simulink model "SigmoidSlidingModeObserver"  (R2026b)
settings: Solver=VariableStepAuto
PostLoadFcn:
  | addpath(fullfile(fileparts(get_param(bdroot,'FileName')),'..','build_process'));initialize_sigmoid_smo_paths();
undefined symbols (not defined in the file or in its folder): sigmoid_smo_parameters, sigmoid_smo_pll_parameters
libraries: AngleTracking x1
settings Model: Creator=24322  LastModifiedBy=24322

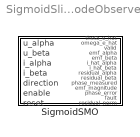
== system SigmoidSlidingModeObserver ==
  SigmoidSMO : Subsystem  mask{cfg=sigmoid_smo_parameters(), trackerCfg=sigmoid_smo_pll_parameters()}
      mask prompts: cfg "Sigmoid SMO configuration"; trackerCfg "PLL configuration"

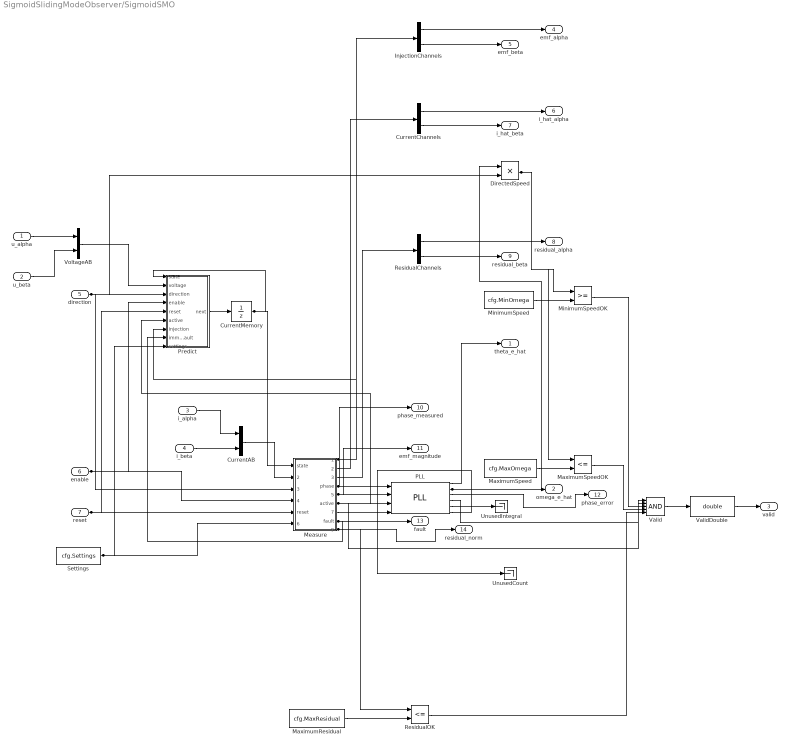
== system SigmoidSlidingModeObserver/SigmoidSMO ==
  u_alpha : Inport  SampleTime=cfg.Ts
  u_beta : Inport  Port=2  SampleTime=cfg.Ts
  i_alpha : Inport  Port=3  SampleTime=cfg.Ts
  i_beta : Inport  Port=4  SampleTime=cfg.Ts
  direction : Inport  Port=5  SampleTime=cfg.Ts
  enable : Inport  Port=6  SampleTime=cfg.Ts
  reset : Inport  Port=7  SampleTime=cfg.Ts
  CurrentAB : Mux  Inputs=2
  CurrentChannels : Demux  Outputs=2
  CurrentMemory : UnitDelay  InitialCondition=zeros(4,1)  SampleTime=cfg.Ts
  DirectedSpeed : Product  Inputs=**
  InjectionChannels : Demux  Outputs=2
  MaximumResidual : Constant  Value=cfg.MaxResidual
  MaximumSpeed : Constant  Value=cfg.MaxOmega
  MaximumSpeedOK : RelationalOperator  Operator=<=  OutDataTypeStr=boolean  RndMeth=Simplest  InputSameDT=off
  Measure : MATLAB Function  TreatAsAtomicUnit=on
  MinimumSpeed : Constant  Value=cfg.MinOmega
  MinimumSpeedOK : RelationalOperator  OutDataTypeStr=boolean  RndMeth=Simplest  InputSameDT=off
  PLL : AngleTracking/PLL  pllCfg=trackerCfg
  Predict : MATLAB Function  TreatAsAtomicUnit=on
  ResidualChannels : Demux  Outputs=2
  ResidualOK : RelationalOperator  Operator=<=  OutDataTypeStr=boolean  RndMeth=Simplest  InputSameDT=off
  Settings : Constant  Value=cfg.Settings
  UnusedCount : Terminator
  UnusedIntegral : Terminator
  Valid : Logic  Inputs=5  IconShape=distinctive  AllPortsSameDT=off  OutDataTypeStr=boolean
  ValidDouble : DataTypeConversion  OutDataTypeStr=double  SaturateOnIntegerOverflow=off  RndMeth=Floor
  VoltageAB : Mux  Inputs=2
  theta_e_hat : Outport
  omega_e_hat : Outport  Port=2
  valid : Outport  Port=3
  emf_alpha : Outport  Port=4
  emf_beta : Outport  Port=5
  i_hat_alpha : Outport  Port=6
  i_hat_beta : Outport  Port=7
  residual_alpha : Outport  Port=8
  residual_beta : Outport  Port=9
  phase_measured : Outport  Port=10
  emf_magnitude : Outport  Port=11
  phase_error : Outport  Port=12
  fault : Outport  Port=13
  residual_norm : Outport  Port=14
  wires:
  ResidualChannels/2 -> residual_beta/1
  ResidualChannels/1 -> residual_alpha/1
  CurrentChannels/2 -> i_hat_beta/1
  CurrentChannels/1 -> i_hat_alpha/1
  InjectionChannels/2 -> emf_beta/1
  InjectionChannels/1 -> emf_alpha/1
  PLL/6 -> UnusedCount/1
  PLL/5 -> UnusedIntegral/1
  PLL/4 -> Valid/1
  PLL/3 -> phase_error/1
  PLL/2 -> DirectedSpeed/1, omega_e_hat/1
  PLL/1 -> theta_e_hat/1
  Measure/9(residualNorm) -> residual_norm/1, ResidualOK/1
  Measure/8(fault) -> Predict/8(immediateFault), fault/1
  Measure/7(trackerReset) -> PLL/4
  Measure/6(active) -> Predict/6(active), Valid/2, PLL/3
  Measure/5(magnitude) -> PLL/2, emf_magnitude/1
  Measure/4(phase) -> PLL/1, phase_measured/1
  Measure/3(residual) -> ResidualChannels/1
  Measure/2(currentHat) -> CurrentChannels/1
  Measure/1(injection) -> Predict/7(injection), InjectionChannels/1
  Predict/1(next) -> CurrentMemory/1
  ValidDouble/1 -> valid/1
  Valid/1 -> ValidDouble/1
  ResidualOK/1 -> Valid/5
  MaximumSpeedOK/1 -> Valid/4
  MinimumSpeedOK/1 -> Valid/3
  MaximumResidual/1 -> ResidualOK/2
  MaximumSpeed/1 -> MaximumSpeedOK/2
  MinimumSpeed/1 -> MinimumSpeedOK/2
  DirectedSpeed/1 -> MinimumSpeedOK/1, MaximumSpeedOK/1
  VoltageAB/1 -> Predict/2(voltage)
  Settings/1 -> Measure/6(settings), Predict/9(settings)
  reset/1 -> Measure/5(reset), Predict/5(reset)
  enable/1 -> Measure/4(enable), Predict/4(enable)
  direction/1 -> DirectedSpeed/2, Measure/3(direction), Predict/3(direction)
  CurrentAB/1 -> Measure/2(current)
  CurrentMemory/1 -> Measure/1(state), Predict/1(state)
  i_beta/1 -> CurrentAB/2
  i_alpha/1 -> CurrentAB/1
  u_beta/1 -> VoltageAB/2
  u_alpha/1 -> VoltageAB/1

== matlab function SigmoidSlidingModeObserver/SigmoidSMO/Predict ==
  data: state input; next output; voltage input; direction input; enable input; reset input; active input; injection input; immediateFault input; settings input
function next=sigmoid_smo_predict(state,voltage,direction,enable,reset,active,injection,immediateFault,settings)
%SIGMOID_SMO_PREDICT Advance current state with this interval's voltage only.
%#codegen
next=zeros(4,1,'like',state);s=cast(settings,'like',state);
if (isfinite(reset) && reset>.5) || (isfinite(enable) && enable<.5),return;end
if immediateFault>0,next(4)=immediateFault;return;end
if state(4)>0,next(4)=state(4);return;end
if direction==0,return;end
next(3)=cast(direction,'like',state);
if active<.5,return;end
u=cast(voltage,'like',state);
if ~all(isfinite(u)) || any(abs(u)>s(5)),next(4)=1;return;end
prediction=s(1)*state(1:2)+s(2)*(u-injection);
if ~all(isfinite(prediction)) || any(abs(prediction)>s(7)),next(4)=3;return;end
next(1:2)=prediction;
end

== matlab function SigmoidSlidingModeObserver/SigmoidSMO/Measure ==
  data: state input; injection output; current input; direction input; enable input; reset input; settings input; currentHat output; residual output; phase output; magnitude output; active output; trackerReset output; fault output; residualNorm output
function [injection,currentHat,residual,phase,magnitude,active,trackerReset,fault,residualNorm]=sigmoid_smo_measure(state,current,direction,enable,reset,settings)
%SIGMOID_SMO_MEASURE Smooth current-error injection; no applied voltage input.
% State=[prior estimated current(2);previous direction;latched fault].
% Settings=[A;B;SlidingGain;Slope;MaxVoltage;MaxCurrent;MaxEstimate].
%#codegen
s=cast(settings,'like',state);injection=zeros(2,1,'like',state);currentHat=injection;residual=injection;
phase=cast(0,'like',state);magnitude=phase;active=phase;trackerReset=cast(1,'like',state);fault=phase;residualNorm=phase;
if (isfinite(reset) && reset>.5) || (isfinite(enable) && enable<.5),return;end
if ~all(isfinite(s)) || s(1)<=0 || s(1)>1 || any(s(2:7)<=0) || ...
        ~isfinite(enable) || ~isfinite(reset) || ~isfinite(direction) || (direction~=0 && abs(direction)~=1)
    fault=cast(2,'like',state);return;
end
if ~all(isfinite(state)),fault=cast(3,'like',state);return;end
if state(4)>0,fault=state(4);return;end
if direction==0 || direction~=state(3),return;end
i=cast(current,'like',state);
if ~all(isfinite(i)) || any(abs(i)>s(6)),fault=cast(1,'like',state);return;end
currentHat=state(1:2);residual=currentHat-i;
injection=s(3)*tanh((s(4)/2)*residual);
phase=atan2(-direction*injection(1),direction*injection(2));
magnitude=hypot(injection(1),injection(2));residualNorm=hypot(residual(1),residual(2));
active=cast(1,'like',state);trackerReset=cast(0,'like',state);
end
